simulink model "gmp_pmsm_sensored_nonlinear_sil_mdl_2022b"  (R2022b)
settings: Solver=VariableStepAuto  StartTime=0.0  StopTime=10  RelTol=1e-3
model workspace (MAT data in the model file):
  B = 0
  BW_i = 800
  Flux_t = 0.12
  IQ24 = Simulink.NumericType
  IQ24.DataTypeMode = 'Fixed-point: binary point scaling'
  IQ24.SignednessBool = 1
  IQ24.WordLength = 32
  IQ24.FixedExponent = -16
  IQ24.SlopeAdjustmentFactor = 1
  IQ24.Bias = 0
  IQ24.DataTypeOverride = 'Inherit'
  IQ24.IsAlias = 0
  IQ24.DataScope = 'Auto'
  J = 0.018
  K_d = 3.72061852168
  K_m = 0.128242020589
  K_u = 0.00236407598332
  Ki_id = 0.001
  Ki_iq = 1
  Ki_n = 25225.1136556
  Kp_id = 1e-05
  Kp_iq = 5e-05
  Kp_n = 12.6125568278
  Ld_t = 0.00303
  Lq_t = 0.02019
  Max_p = 0.006000830667
  P = 2
  RLS_ini_a = 1000000
  Rd_mos = 0.01
  Rs = 0.1215
  Rv = 6.4
  T_final = 0
  T_initial = 0
  Tes = [4 7 10 7 4]
  Tf_t = 0.1
  Tm = 0
  Udq_limit = 550
  Var = 0
  Vce0 = 0
  Vd0 = 0
  Vdc = 80
  button = 1
  im_limit = 40
  mean_prd = 10
  position_init = 0.2
  r_ce = 1e-08
  r_d = 1e-08
  sample_prd = 100
  step_time = 0.2
  ts = 6.25e-05
  wc = 3500
libraries: peripheral_utilities x9, spsSeriesRLCBranchLib x6, spsMosfetLib x6, simulink x3, spsVoltageMeasurementLib x2, gmp_sil_core_pack x1, spsPermanentMagnetSynchronousMachineLib x1, spsdq0toabcLib x1, spsFourierLib x1, spsControlledVoltageSourceLib x1, sps_lib x1
(part 1 of 3)
settings Model: SimulationMode=accelerator  Creator=javnson  LastModifiedBy=Lin Minyi

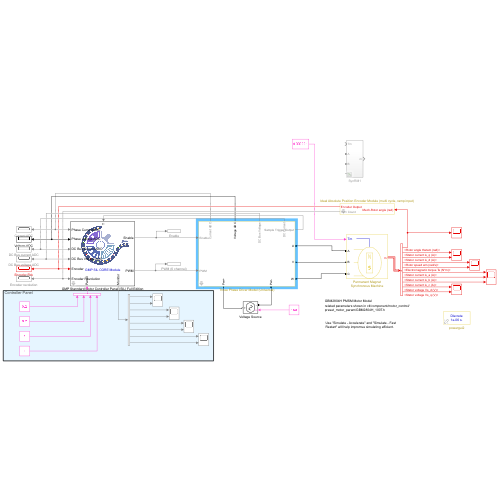
[thumbnail: Simulink's stored preview of the top-level diagram]
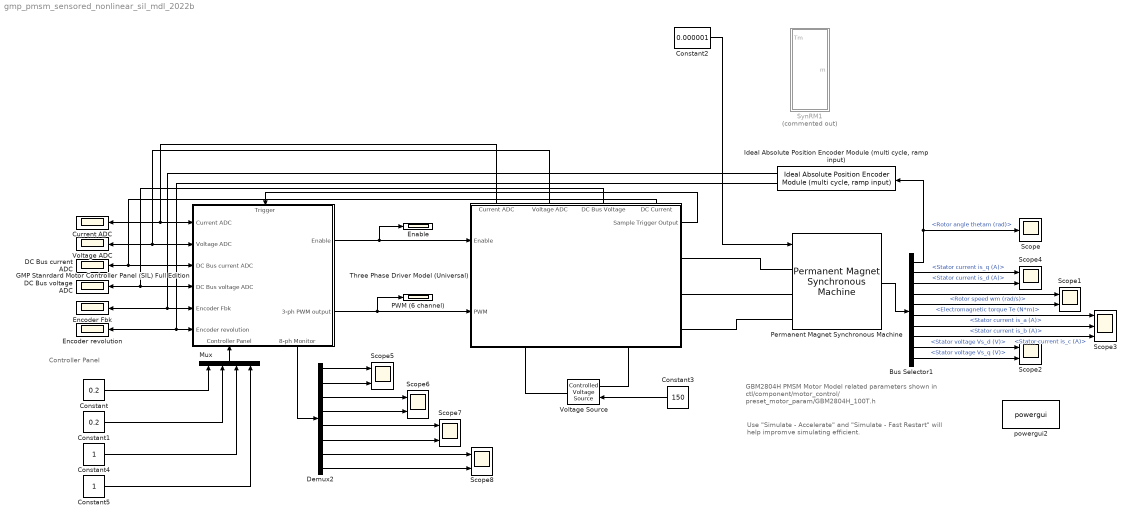
== system gmp_pmsm_sensored_nonlinear_sil_mdl_2022b ==
  note: Use "Simulate - Accelerate" and "Simulate - Fast Restart" will help impromve simulating efficient.
  note: Controller Panel
  note: GBM2804H PMSM Motor Model
      | related parameters shown in ctl/component/motor_control/
      | preset_motor_param/GBM2804H_100T.h
  Bus Selector1 : BusSelector  OutputSignals=Rotor angle thetam (rad),Stator current is_q (A),Stator current is_d (A),Rotor speed wm (rad/s),Electromagnetic torque Te (N*m),Stator current is_a (A),Stator current is_b (A),Stator current is_c (A),Stator voltage Vs_d (V),Stator voltage Vs_q (V)
  Constant : Constant  Value=0.2
  Constant1 : Constant  Value=0.2
  Constant2 : Constant  Value=0.000001
  Constant3 : Constant  Value=150
  Constant4 : Constant
  Constant5 : Constant
  Current ADC : Scope
  DC Bus current ADC : Scope
  DC Bus voltage ADC : Scope
  Demux2 : Demux  Outputs=8
  Enable : Scope
  Encoder Fbk : Scope
  Encoder revolution : Scope
  GMP Stanrdard Motor Controller Panel (SIL) Full Edition : Subsystem  mask(GMP SIL Core for single Motor Controller (full edition)){}
      mask help: This is GMP Motor Simulator port.
      settings: PortSchema="{\"entries\":[{\"content\":{\"sides\":[{\"content\":{\"connectorIds\":[\"In1\",\"In2\",\"In3\",\"In4\",\"In5\",\"In6\"]},\"type\":\"ConnectorPlacement.EquallySpacedRectSide\",\"uuid\":\"45c67bc9-9540-469a-a4ac-1e12eb9acca3\"},{\"content\":{\"connectorIds\":[\"Out1\",\"Out2\"],\"side\":\"RIGHT\"},\"type\":\"ConnectorPlacement.EquallySpacedRectSide\",\"uuid\":\"a17116b4-0460-48ab-8ada-a785da6c5e29\"},{\"content\":{\"connectorIds\":[\"In7\"],\"side\":\"TOP\"},\"type\":\"ConnectorPlacement.EquallySpacedRectSide\",\"uuid\":\"15623697-512e-4e4d-ab51-f53c2346fadb\"},{\"content\":{\"connectorIds\":[\"In8\",\"Out3\"],\"side\":\"BOTTOM\"},\"type\":\"ConnectorPlacement.EquallySpacedRectSide\",\"uuid\":\"47f7968c-22c1-4f3d-97d9-242e9dbf8d30\"}]},\"type\":\"ConnectorPlacement.EquallySpacedConnector\",\"uuid\":\"f369880c-e675-4c1f-982e-a4befb03f503\"}],\"packageUris\":[\"http://schema.mathworks.com/mf0/Connector/R2020b\"],\"version\":\"1.0\"}"
      mask DialogControl ParameterGroupVar Prompt: 参数
      mask Display:
      | image(append(fileparts(which('gmp_simulink_utilities.slx')),'\icon\GMP_Core.png'));
      | color('blue');
      | %text(0.3,0.3,'GMP SIL CORE Module','horizontalAlignment','left','verticalAlignment','bottom');
      | disp('\n\n\n\n\n\n\n\nGMP SIL CORE Module');
      | %text(0,0,'y=a*x^2+b','horizontalAlignment','middle', 'verticalAlignment','bottom');
      | 
      | 
      | module_pos = get_param(gcb, 'Position');
      | width = module_pos(3) - module_pos(1);
      | %rectangle('Position',[module_pos(1),module_pos(2),module_pos(3),module_pos(4)],'FaceColor','r');
      | 
      | color('Black');
      | 
      | port_label('output', 1, 'Enable');
      | port_label('output', 2, 'PWM');
      | port_label('output', 3, 'Monitor');
      | 
      | port_label('input', 1, 'Phase Current ADC');
      | port_label('input', 2, 'Phase Voltage ADC');
      | port_label('input', 3, 'DC Bus Current ADC');
      | port_label('input', 4, 'DC Bus Voltage ADC');
      | port_label('input', 5, 'Encoder');
      | port_label('input', 6, 'Encoder Revolution');
      | port_label('input', 7, 'T');
      | port_label('input', 8, 'Panel');
  "Ideal Absolute Position Encoder Module (multi cycle, ramp input)" : peripheral_utilities/Ideal Absolute Position Encoder Module (multi cycle, ramp input)  ENCODER_BIT=14
      settings: SourceProductName=GMP Utilities Library
  Mux : Mux
  PWM (6 channel) : Scope
  Permanent Magnet Synchronous Machine : spsPermanentMagnetSynchronousMachineLib/Permanent Magnet Synchronous Machine  NbPhases=3  FluxDistribution=Sinusoidal  RotorType=Salient-pole  MechanicalLoad=Torque Tm  PresetModel=No  ShowDetailedParameters=on  MeasurementBus=off  Resistance=Rs  Inductance=8.5e-3  dqInductances=[Ld_t,Lq_t]  La=0.96e-3  MachineConstant=Flux linkage established by magnets (V.s)  Flux=Flux_t  VoltageCst=43.5312  TorqueCst=0.36  Flat=120  Mechanical=[J 1e-8 P 0]  PolePairs=4  InitialConditions=[0, 0, 0, 0]  InitialConditions5ph=[0 0 0 0 0 0]  RefAngle=Aligned with phase A axis (original Park)  IterativeDiscreteModel=Trapezoidal non iterative  TsBlock=-1  TsPowergui=0
  Scope : Scope
  Scope{1..2,4..8} (7 alike) : Scope  NumInputPorts=2
  Scope3 : Scope  NumInputPorts=3
  SynRM1 : Subsystem  Commented=on
  Three Phase Driver Model (Universal) : Subsystem  mask{fswitch=8000, CMP_MAX=6000, Deadband_Upper=48, Deadband_Lower=48, Deadband_us=1, phase_shift=0, R_mosfet_on=0.1, Lon=0, Rd=0.01, Vf=0.3, Rs=1e5, Cs=inf, Rsap=0.005, ADC_GAIN=20, ADC_BIT=12, ADC_REFERENCE=3.3, ADC_BIAS=1.65, ADC_INIT=0, VOLTAGE_ADC_GAIN=0.04049127, VOLTAGE_ADC_BIT=12, VOLTAGE_ADC_REFERENCE=3.3, VOLTAGE_ADC_VOLTAGE=0, VOLTAGE_ADC_INIT=0, VOLTAGE_ADC_CUT_FREQ=1143.4, DCBUS_ADC_GAIN=0.04049127, DCBUS_ADC_BIT=12, DCBUS_ADC_REFERENCE=3.3, DCBUS_ADC_BIAS=0, DCBUS_ADC_INIT=0, DCBUS_CURRENT_ADC_GAIN=1, DCBUS_CURRENT_ADC_BIT=12, DCBUS_CURRENT_ADC_REFERENCE=20, DCBUS_CURRENT_ADC_BIAS=0, DCBUS_CURRENT_ADC_INIT=0}
      mask prompts: DCBUS_CURRENT_ADC_GAIN "DCBUS_ADC_GAIN:"; DCBUS_CURRENT_ADC_BIT "DCBUS_ADC_BIT:"; DCBUS_CURRENT_ADC_REFERENCE "DCBUS_ADC_REFERENCE:"; DCBUS_CURRENT_ADC_BIAS "DCBUS_ADC_BIAS:"; DCBUS_CURRENT_ADC_INIT "DCBUS_ADC_INIT:"
      mask init:
      | calculate_deadband(gcb, 'Deadband_Upper', 'Deadband_Lower',	'CMP_MAX', 'fswitch', 'Deadband_us');
      settings: PortSchema="{\"entries\":[{\"content\":{\"sides\":[{\"content\":{\"connectorIds\":[\"In1\",\"In2\"]},\"type\":\"ConnectorPlacement.EquallySpacedRectSide\",\"uuid\":\"3f4c86ad-0582-4f47-8583-a8af9a7f9adc\"},{\"content\":{\"connectorIds\":[\"Out1\",\"RConn1\",\"RConn2\",\"RConn3\"],\"side\":\"RIGHT\"},\"type\":\"ConnectorPlacement.EquallySpacedRectSide\",\"uuid\":\"ae91f325-3014-4188-9063-296f4d5623fa\"},{\"content\":{\"connectorIds\":[\"Out2\",\"Out3\",\"Out4\",\"Out5\"],\"side\":\"TOP\"},\"type\":\"ConnectorPlacement.EquallySpacedRectSide\",\"uuid\":\"5f2edb36-6849-4a72-b7bd-4d267f120ce4\"},{\"content\":{\"connectorIds\":[\"RConn4\",\"RConn5\"],\"side\":\"BOTTOM\"},\"type\":\"ConnectorPlacement.EquallySpacedRectSide\",\"uuid\":\"79a111ed-6591-4ced-9242-67ea1247c580\"}]},\"type\":\"ConnectorPlacement.EquallySpacedConnector\",\"uuid\":\"8c66eb8e-d25c-472f-a4a5-d1759225ba1c\"}],\"packageUris\":[\"http://schema.mathworks.com/mf0/Connector/R2020b\"],\"version\":\"1.0\"}"
      mask Callback fswitch: calculate_deadband(gcb, 'Deadband_Upper', 'Deadband_Lower',	'CMP_MAX', 'fswitch', 'Deadband_us');
      mask Callback CMP_MAX: calculate_deadband(gcb, 'Deadband_Upper', 'Deadband_Lower',	'CMP_MAX', 'fswitch', 'Deadband_us');
      mask Callback Deadband_Upper: calculate_deadband(gcb, 'Deadband_Upper', 'Deadband_Lower',	'CMP_MAX', 'fswitch', 'Deadband_us');
      mask Callback Deadband_Lower: calculate_deadband(gcb, 'Deadband_Upper', 'Deadband_Lower',	'CMP_MAX', 'fswitch', 'Deadband_us');
      mask DialogControl DescGroupVar Prompt: Three Phases Bridge Peripheral(3-shunt sample)
      mask DialogControl Control21 Prompt: GMP CTL Simulink Utilities: virtual peripherals
      mask DialogControl DescTextVar Prompt: This module provide a ideal 3-phases bridge peripheral.
      mask DialogControl Container4 Prompt: PWM config
      mask DialogControl ParameterGroupVar Prompt: PWM parameters
      mask DialogControl Control2 Prompt: PWM Frequency (Hz):
      mask DialogControl Control4 Prompt: Full Scale PWM Compare value:
      mask DialogControl Control5 Prompt: Deadband Range Set (CMP Value):
      mask DialogControl Control6 Prompt: Deadband time: DEADBAND_CMP/2/CMP_MAX/fswitch
      mask DialogControl Control22 Prompt: Calculated Deadband, us
      mask DialogControl Control20 Prompt: Initial Phase shift:
      mask DialogControl Container5 Prompt: MOSFET config
      mask DialogControl Container7 Prompt: MOSFET parameters
      mask DialogControl Control7 Prompt: Rds(on), unit Ohm
      mask DialogControl Control8 Prompt: Internal diode inducctance, unit H
      mask DialogControl Control9 Prompt: Internal diode resistance Rd, unit Ohm
      mask DialogControl Control10 Prompt: Internal diode forward voltage Vf, unit V
      mask DialogControl Control11 Prompt: Snubber resistance Rs, unit ohm
      mask DialogControl Control12 Prompt: Snubber Capacitance Cs, unit F
      mask DialogControl Container6 Prompt: 3-shunt Current Sample
      mask DialogControl Control13 Prompt: ADC(p.u.) = (real_voltage * ADC_GAIN + ADC_BIAS)/ADC_REFERENCE
      mask DialogControl Control15 Prompt: Shunt Smaple Res, unit Ohm
      mask DialogControl Control14 Prompt: ADC Voltage Gain (Scale Factor):
      mask DialogControl Control16 Prompt: ADC resolution:
      mask DialogControl Control17 Prompt: ADC reference Voltage(V)
      mask DialogControl Control18 Prompt: ADC Bias Voltage(V)
      mask DialogControl Control19 Prompt: ADC Initial Voltage Output (V):
      mask DialogControl Container9 Prompt: 3-shunt Voltage Sample
      mask DialogControl Control34 Prompt: ADC Voltage Gain (Scale Factor):
      mask DialogControl Control23 Prompt: ADC resolution:
      mask DialogControl Control24 Prompt: ADC reference voltage (V), when VOLTAGE_ADC_GAIN = 1, ADC_REF = ADC Full scale
      mask DialogControl Control25 Prompt: ADC Bias Voltage (V):
      mask DialogControl Control26 Prompt: ADC Initial Voltage Output (V):
      mask DialogControl Control27 Prompt: Voltage Filter cut frequency (Hz):
      mask DialogControl Control28 Prompt: Generally, this value less than switch frequency / 10, greater than motor normal frequency * 3
      mask DialogControl Container10 Prompt: DC Bus Voltage Sample
      mask DialogControl Control29 Prompt: ADC Voltage Gain (Scale Factor):
      mask DialogControl Control30 Prompt: ADC resolution:
      mask DialogControl Control32 Prompt: ADC reference voltage (V), when VOLTAGE_ADC_GAIN = 1, ADC_REF = ADC Full scale
      mask DialogControl Control31 Prompt: ADC Bias Voltage (V):
      mask DialogControl Control33 Prompt: ADC Initial Voltage Output (V):
      mask DialogControl Container13 Prompt: DC Bus Current Sample
      mask DialogControl Control29_copy_copy Prompt: ADC Current Gain (Scale Factor):
      mask DialogControl Control30_copy_copy Prompt: ADC resolution:
      mask DialogControl Control32_copy_copy Prompt: ADC reference current (A), when VOLTAGE_ADC_GAIN = 1, ADC_REF = ADC Full scale
      mask DialogControl Control31_copy Prompt: ADC Bias Current (A):
      mask DialogControl Control33_copy Prompt: ADC Initial Current Output (A):
  Voltage ADC : Scope
  Voltage Source : spsControlledVoltageSourceLib/Controlled Voltage Source  Initialize=on  Source_Type=AC  Amplitude=0  Phase=0  Frequency=0  Measurements=None
  powergui2 : sps_lib/powergui  Priority=1  SimulationMode=Discrete  SampleTime=1e-6  frequency=60  Iterations=50  frequencyindice=0  Pbase=100e6  ErrMax=1e-4  UnitsV=kV  UnitsW=MW  buscounter=0  FunctionMessages=off  echomessages=off  EnableUseOfTLC=off  CurrentSourceSwitches=off  DisableSnubberDevices=off  DisableRonSwitches=off  DisableVfSwitches=off  DisplayEquations=off  AutomaticDiscreteSolvers=off  SolverType=Tustin/Backward Euler (TBE)  Interpol=off  ExternalGateDelay=off  methode=off  Ts=100  x0status=blocks  SPID=on  SwTol=0  HookPort=off  NonlinearTolerance=1e-4  nMaxIteration=100  ContinueOnMaxIteration=off  RestoreLinks=warning  ResistiveCurrentMeasurement=off  Frange=[0:2:500]  Ylog=off  Xlog=on  ShowGrid=off  save=off  variable=ZData  structure=0  ZoomFFT=off  StartTime=0.0  cycles=1  DisplayStyle=1  fundamental=60  FreqAxis=off  MaxFrequency=1000  frequencyindicesteady=1  RmsSteady=1  display=off
  wires:
  GMP Stanrdard Motor Controller Panel (SIL) Full Edition/1(Enable) -> Three Phase Driver Model (Universal)/1(Enable), Enable/1
  GMP Stanrdard Motor Controller Panel (SIL) Full Edition/2(3-ph PWM output) -> PWM (6 channel)/1, Three Phase Driver Model (Universal)/2(PWM)
  Constant2/1 -> Permanent Magnet Synchronous Machine/1
  Three Phase Driver Model (Universal)/1(Sample Trigger Output) -> GMP Stanrdard Motor Controller Panel (SIL) Full Edition/7(Trigger)
  Three Phase Driver Model (Universal)/2(Current ADC) -> GMP Stanrdard Motor Controller Panel (SIL) Full Edition/1(Current ADC), Current ADC/1
  Three Phase Driver Model (Universal)/3(Voltage ADC) -> GMP Stanrdard Motor Controller Panel (SIL) Full Edition/2(Voltage ADC), Voltage ADC/1
  Three Phase Driver Model (Universal)/4(DC Bus Voltage) -> DC Bus voltage ADC/1, GMP Stanrdard Motor Controller Panel (SIL) Full Edition/4(DC Bus voltage ADC)
  Permanent Magnet Synchronous Machine/1 -> Bus Selector1/1
  Bus Selector1/1 -> "Ideal Absolute Position Encoder Module (multi cycle, ramp input)"/1, Scope/1  "<Rotor angle thetam (rad)>"
  "Ideal Absolute Position Encoder Module (multi cycle, ramp input)"/1 -> Encoder Fbk/1, GMP Stanrdard Motor Controller Panel (SIL) Full Edition/5(Encoder Fbk)
  Bus Selector1/3 -> Scope4/2  "<Stator current is_d (A)>"
  Bus Selector1/2 -> Scope4/1  "<Stator current is_q (A)>"
  Constant3/1 -> Voltage Source/1
  Demux2/4 -> Scope6/2
  Demux2/3 -> Scope6/1
  Demux2/2 -> Scope5/2
  Demux2/1 -> Scope5/1
  GMP Stanrdard Motor Controller Panel (SIL) Full Edition/3(8-ph Monitor) -> Demux2/1
  Bus Selector1/4 -> Scope1/1  "<Rotor speed wm (rad/s)>"
  Bus Selector1/5 -> Scope1/2  "<Electromagnetic torque Te (N*m)>"
  "Ideal Absolute Position Encoder Module (multi cycle, ramp input)"/2 -> Encoder revolution/1, GMP Stanrdard Motor Controller Panel (SIL) Full Edition/6(Encoder revolution)
  Mux/1 -> GMP Stanrdard Motor Controller Panel (SIL) Full Edition/8(Controller Panel)
  Constant/1 -> Mux/1
  Constant1/1 -> Mux/2
  Constant4/1 -> Mux/3
  Constant5/1 -> Mux/4
  Demux2/5 -> Scope7/1
  Demux2/6 -> Scope7/2
  Demux2/7 -> Scope8/1
  Demux2/8 -> Scope8/2
  Three Phase Driver Model (Universal)/5(DC Current) -> DC Bus current ADC/1, GMP Stanrdard Motor Controller Panel (SIL) Full Edition/3(DC Bus current ADC)
  Bus Selector1/9 -> Scope2/1  "<Stator voltage Vs_d (V)>"
  Bus Selector1/10 -> Scope2/2  "<Stator voltage Vs_q (V)>"
  Bus Selector1/6 -> Scope3/1  "<Stator current is_a (A)>"
  Bus Selector1/7 -> Scope3/2  "<Stator current is_b (A)>"
  Bus Selector1/8 -> Scope3/3  "<Stator current is_c (A)>"
  connections:
  Permanent Magnet Synchronous Machine/LConn2 -- Three Phase Driver Model (Universal)/RConn2
  Three Phase Driver Model (Universal)/RConn3 -- Permanent Magnet Synchronous Machine/LConn3
  Permanent Magnet Synchronous Machine/LConn1 -- Three Phase Driver Model (Universal)/RConn1
  Three Phase Driver Model (Universal)/RConn5 -- Voltage Source/LConn1
  Three Phase Driver Model (Universal)/RConn4 -- Voltage Source/RConn1

== system gmp_pmsm_sensored_nonlinear_sil_mdl_2022b/GMP Stanrdard Motor Controller Panel (SIL) Full Edition ==
  Current ADC : Inport
  Voltage ADC : Inport  Port=2
  DC Bus current ADC : Inport  Port=3
  DC Bus voltage ADC : Inport  Port=4
  Encoder Fbk : Inport  Port=5
  Encoder revolution : Inport  Port=6
  Trigger : Inport  Port=7
  Controller Panel : Inport  Port=8
  GMP SIL Core With trigger : Subsystem
  Simulation Time : Clock
  Enable : Outport
  3-ph PWM output : Outport  Port=2
  8-ph Monitor : Outport  Port=3
  wires:
  Encoder Fbk/1 -> GMP SIL Core With trigger/6(Encoder Fbk)
  Encoder revolution/1 -> GMP SIL Core With trigger/7(Encoder revolution)
  GMP SIL Core With trigger/2(3-ph PWM output) -> 3-ph PWM output/1
  Simulation Time/1 -> GMP SIL Core With trigger/1(time)
  GMP SIL Core With trigger/1(Enable) -> Enable/1
  Voltage ADC/1 -> GMP SIL Core With trigger/3(Voltage ADC)
  Current ADC/1 -> GMP SIL Core With trigger/2(Current ADC)
  GMP SIL Core With trigger/3(8-ph Monitor) -> 8-ph Monitor/1
  DC Bus current ADC/1 -> GMP SIL Core With trigger/4(DC Bus current ADC)
  Trigger/1 -> GMP SIL Core With trigger/Trigger
  DC Bus voltage ADC/1 -> GMP SIL Core With trigger/5(DC bus voltage ADC)
  Controller Panel/1 -> GMP SIL Core With trigger/8(Panel Input)

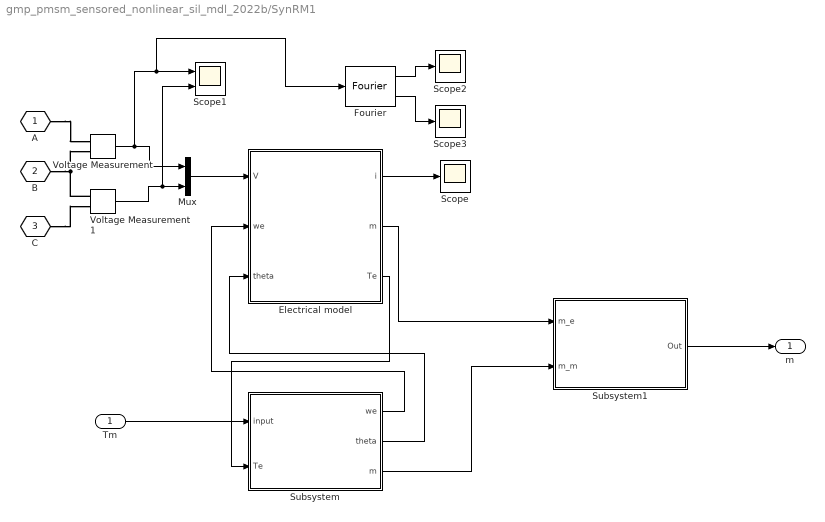
== system gmp_pmsm_sensored_nonlinear_sil_mdl_2022b/SynRM1 ==
  Tm : Inport
  Electrical model : Subsystem
  Fourier : spsFourierLib/Fourier  Freq=100  n=1  InInit=[0, 0]  Ts=0
  Mux : Mux  Inputs=2
  Scope : Scope
  Scope1 : Scope  NumInputPorts=2
  Scope2 : Scope
  Scope3 : Scope
  Subsystem : Subsystem
  Subsystem1 : Subsystem
  Voltage Measurement : spsVoltageMeasurementLib/Voltage Measurement  PhasorSimulation=off  OutputType=Complex  PSBequivalent=0
  Voltage Measurement1 : spsVoltageMeasurementLib/Voltage Measurement  PhasorSimulation=off  OutputType=Complex  PSBequivalent=0
  A : PMIOPort  Side=Left
  B : PMIOPort  Port=2  Side=Left
  C : PMIOPort  Port=3  Side=Left
  m : Outport  VectorParamsAs1DForOutWhenUnconnected=off
  wires:
  Subsystem/3(m) -> Subsystem1/2(m_m)
  Subsystem/1(we) -> Electrical model/2(we)
  Mux/1 -> Electrical model/1(V)
  Subsystem/2(theta) -> Electrical model/3(theta)
  Electrical model/3(Te) -> Subsystem/2(Te)
  Subsystem1/1(Out) -> m/1
  Electrical model/1(i) -> Scope/1
  Electrical model/2(m) -> Subsystem1/1(m_e)
  Tm/1 -> Subsystem/1(input)
  Voltage Measurement/1 -> Fourier/1, Scope1/1, Mux/1
  Voltage Measurement1/1 -> Scope1/2, Mux/2
  Fourier/1 -> Scope2/1
  Fourier/2 -> Scope3/1
  connections:
  C/RConn1 -- Voltage Measurement1/LConn2
  A/RConn1 -- Voltage Measurement/LConn1
  B/RConn1 -- Voltage Measurement1/LConn1 -- Voltage Measurement/LConn2

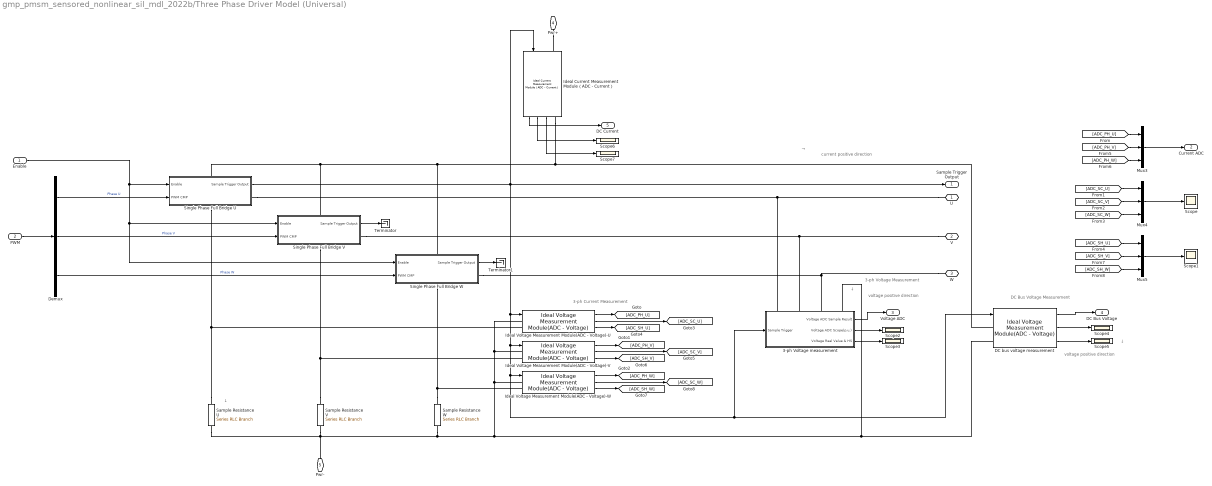
== system gmp_pmsm_sensored_nonlinear_sil_mdl_2022b/Three Phase Driver Model (Universal) ==
  note: 3-ph Current Measurement
  note: →
  note: current positive direction
  note: ↓
  note: voltage positive direction
  note: ↓
  note: 3-ph Voltage Measurement
  note: DC Bus Voltage Measurement
  note: ↓
  note: voltage positive direction
  Enable : Inport
  PWM : Inport  Port=2
  3-ph Voltage measurement : Subsystem  AncestorBlock=peripheral_utilities/Three Phases Voltage (ph-gnd) Measurement with Filter  mask{ADC_GAIN=VOLTAGE_ADC_GAIN, ADC_BIT=VOLTAGE_ADC_BIT, ADC_REFERENCE=VOLTAGE_ADC_REFERENCE, ADC_BIAS=VOLTAGE_ADC_VOLTAGE, ADC_INIT=VOLTAGE_ADC_INIT, cut_frequency=VOLTAGE_ADC_CUT_FREQ}
      settings: PortSchema="{\"entries\":[{\"content\":{\"sides\":[{\"content\":{\"connectorIds\":[\"In1\"]},\"type\":\"ConnectorPlacement.EquallySpacedRectSide\",\"uuid\":\"ae4f4612-c092-4fa0-8a43-5c9e823110e3\"},{\"content\":{\"connectorIds\":[\"Out1\",\"Out2\",\"Out3\"],\"side\":\"RIGHT\"},\"type\":\"ConnectorPlacement.EquallySpacedRectSide\",\"uuid\":\"6db15ef0-d33a-4775-b4e6-14a566796673\"},{\"content\":{\"connectorIds\":[\"LConn1\",\"LConn2\",\"LConn3\",\"LConn4\"],\"side\":\"TOP\"},\"type\":\"ConnectorPlacement.EquallySpacedRectSide\",\"uuid\":\"cfddd664-59f3-497b-b33e-fe832fe7a7bd\"}]},\"type\":\"ConnectorPlacement.EquallySpacedConnector\",\"uuid\":\"5bacf0ad-0c4a-4f47-a242-d8a476ab7f52\"}],\"packageUris\":[\"http://schema.mathworks.com/mf0/Connector/R2020b\"],\"version\":\"1.0\"}"
      mask DialogControl DescGroupVar Prompt: 3 phases Voltage Sample ADC Model
      mask DialogControl Control10 Prompt: GMP CTL Simulink Utilities: virtual peripherals
      mask DialogControl DescTextVar Prompt: This is a ideal Voltage Measurement Module.
      mask DialogControl Control2 Prompt: ADC(p.u.) = (real_voltage * ADC_GAIN + ADC_BIAS)/ADC_REFERENCE
      mask DialogControl ParameterGroupVar Prompt: parameters:
      mask DialogControl Control3 Prompt: ADC Voltage Gain (Scale Factor):
      mask DialogControl Control4 Prompt: ADC resolution:
      mask DialogControl Control5 Prompt: ADC reference Voltage (V), when ADC_GAIN=1, ADC_REF = ADC full scale
      mask DialogControl Control6 Prompt: ADC Bias Voltage(V)
      mask DialogControl Control7 Prompt: ADC Initial Voltage Output (V):
      mask DialogControl Control8 Prompt: Voltage Filter cut frequency (Hz):
      mask DialogControl Control9 Prompt: Generally, this value less than switch frequency / 10, greater than motor normal frequency * 3
  DC bus voltage measurement : peripheral_utilities/Ideal Voltage Measurement Module(ADC - Voltage)  ADC_GAIN=DCBUS_ADC_GAIN  ADC_BIT=DCBUS_ADC_BIT  ADC_REFERENCE=DCBUS_ADC_REFERENCE  ADC_BIAS=DCBUS_ADC_BIAS  ADC_INIT=DCBUS_ADC_INIT
      settings: SourceProductName=GMP Utilities Library
  Demux : Demux  Outputs=3
  Ideal Current Measurement Module（ADC - Current） : peripheral_utilities/Ideal Current Measurement Module（ADC - Current）  ADC_GAIN=DCBUS_CURRENT_ADC_GAIN  ADC_BIT=DCBUS_CURRENT_ADC_BIT  ADC_REFERENCE=DCBUS_CURRENT_ADC_REFERENCE  ADC_BIAS=DCBUS_CURRENT_ADC_BIAS  ADC_INIT=DCBUS_CURRENT_ADC_INIT
      settings: SourceProductName=GMP Utilities Library
  Ideal Voltage Measurement Module(ADC - Voltage)-U : peripheral_utilities/Ideal Voltage Measurement Module(ADC - Voltage)  ADC_GAIN=ADC_GAIN  ADC_BIT=ADC_BIT  ADC_REFERENCE=ADC_REFERENCE  ADC_BIAS=ADC_BIAS  ADC_INIT=ADC_INIT
      settings: SourceProductName=GMP Utilities Library
  Ideal Voltage Measurement Module(ADC - Voltage)-V : peripheral_utilities/Ideal Voltage Measurement Module(ADC - Voltage)  ADC_GAIN=ADC_GAIN  ADC_BIT=ADC_BIT  ADC_REFERENCE=ADC_REFERENCE  ADC_BIAS=ADC_BIAS  ADC_INIT=ADC_INIT
      settings: SourceProductName=GMP Utilities Library
  Ideal Voltage Measurement Module(ADC - Voltage)-W : peripheral_utilities/Ideal Voltage Measurement Module(ADC - Voltage)  ADC_GAIN=ADC_GAIN  ADC_BIT=ADC_BIT  ADC_REFERENCE=ADC_REFERENCE  ADC_BIAS=ADC_BIAS  ADC_INIT=ADC_INIT
      settings: SourceProductName=GMP Utilities Library
  Mux3 : Mux  Inputs=3
  Mux4 : Mux  Inputs=3
  Mux5 : Mux  Inputs=3
  Sample Resistance U : spsSeriesRLCBranchLib/Series RLC Branch  LConnTagsString=__new0  RConnTagsString=__new0  BranchType=R  Resistance=Rsap  Inductance=1e-3  SetiL0=off  InitialCurrent=0  Capacitance=1e-6  Setx0=off  InitialVoltage=0  Measurements=None
  Sample Resistance V : spsSeriesRLCBranchLib/Series RLC Branch  LConnTagsString=__new0  RConnTagsString=__new0  BranchType=R  Resistance=Rsap  Inductance=1e-3  SetiL0=off  InitialCurrent=0  Capacitance=1e-6  Setx0=off  InitialVoltage=0  Measurements=None
  Sample Resistance W : spsSeriesRLCBranchLib/Series RLC Branch  LConnTagsString=__new0  RConnTagsString=__new0  BranchType=R  Resistance=Rsap  Inductance=1e-3  SetiL0=off  InitialCurrent=0  Capacitance=1e-6  Setx0=off  InitialVoltage=0  Measurements=None
  Scope{,1..7} (8 alike) : Scope
  Single Phase Full Bridge U : Subsystem  mask{fswitch=fswitch, CMP_MAX=CMP_MAX, Deadband_Upper=Deadband_Upper, Deadband_Lower=Deadband_Lower, Deadband_us=NaN, phase_shift=phase_shift, R_mosfet_on=R_mosfet_on, Lon=Lon, Rd=Rd, Vf=Vf, Rs=Rs, Cs=Cs}
      mask init:
      | calculate_deadband(gcb, 'Deadband_Upper', 'Deadband_Lower',	'CMP_MAX', 'fswitch', 'Deadband_us');
      settings: PortSchema="{\"entries\":[{\"content\":{\"sides\":[{\"content\":{\"connectorIds\":[\"In1\",\"In2\"]},\"type\":\"ConnectorPlacement.EquallySpacedRectSide\",\"uuid\":\"20beeabc-b0ca-4337-b227-c7f02abd15d8\"},{\"content\":{\"connectorIds\":[\"Out1\",\"RConn1\"],\"side\":\"RIGHT\"},\"type\":\"ConnectorPlacement.EquallySpacedRectSide\",\"uuid\":\"a7923383-ac55-4621-ad1d-4d067c1fb84d\"},{\"content\":{\"connectorIds\":[\"LConn1\"],\"side\":\"TOP\"},\"type\":\"ConnectorPlacement.EquallySpacedRectSide\",\"uuid\":\"661bf0ae-1c96-4de8-96aa-28c06a0a56db\"},{\"content\":{\"connectorIds\":[\"RConn2\"],\"side\":\"BOTTOM\"},\"type\":\"ConnectorPlacement.EquallySpacedRectSide\",\"uuid\":\"fc2f6321-5787-4e1a-b5a2-65ed34db36b5\"}]},\"type\":\"ConnectorPlacement.EquallySpacedConnector\",\"uuid\":\"e2219b16-0a50-43ef-8183-c55a35d5a2a0\"}],\"packageUris\":[\"http://schema.mathworks.com/mf0/Connector/R2020b\"],\"version\":\"1.0\"}"
      mask Callback fswitch: calculate_deadband(gcb, 'Deadband_Upper', 'Deadband_Lower',	'CMP_MAX', 'fswitch', 'Deadband_us');
      mask Callback CMP_MAX: calculate_deadband(gcb, 'Deadband_Upper', 'Deadband_Lower',	'CMP_MAX', 'fswitch', 'Deadband_us');
      mask Callback Deadband_Upper: calculate_deadband(gcb, 'Deadband_Upper', 'Deadband_Lower',	'CMP_MAX', 'fswitch', 'Deadband_us');
      mask Callback Deadband_Lower: calculate_deadband(gcb, 'Deadband_Upper', 'Deadband_Lower',	'CMP_MAX', 'fswitch', 'Deadband_us');
      mask DialogControl DescGroupVar Prompt: Half Bridge With PWM Module
      mask DialogControl Control14 Prompt: GMP CTL Simulink Utilities: virtual peripherals
      mask DialogControl DescTextVar Prompt: This module provide a PWM (with deadband), and a MOSFET half bridge.
      mask DialogControl Container5 Prompt: PWM Modulator
      mask DialogControl ParameterGroupVar Prompt: PWM module parameters
      mask DialogControl Control2 Prompt: PWM Frequency (Hz):
      mask DialogControl Control3 Prompt: Full Scale PWM Compare value:
      mask DialogControl Control4 Prompt: (whole period is 2 * CMP_MAX ticks)
      mask DialogControl Control5 Prompt: Deadband Range Set (CMP Value):
      mask DialogControl Control6 Prompt: Single side deadband time: DEADBAND_CMP/2/CMP_MAX/fswitch
      mask DialogControl Control15 Prompt: Calculated Deadband, us
      mask DialogControl Control13 Prompt: Initial Phase Shift, unit rad
      mask DialogControl Container6 Prompt: MOSFET
      mask DialogControl Container3 Prompt: MOSFET parameters
      mask DialogControl Control7 Prompt: Rds(on), unit Ohm
      mask DialogControl Control8 Prompt: Internal diode inducctance, unit H
      mask DialogControl Control9 Prompt: Internal diode resistance Rd, unit Ohm
      mask DialogControl Control10 Prompt: Internal diode forward voltage Vf, unit V
      mask DialogControl Control11 Prompt: Snubber resistance Rs, unit ohm
      mask DialogControl Control12 Prompt: Snubber Capacitance Cs, unit F
  Single Phase Full Bridge V : Subsystem  mask{fswitch=fswitch, CMP_MAX=CMP_MAX, Deadband_Upper=Deadband_Upper, Deadband_Lower=Deadband_Lower, Deadband_us=NaN, phase_shift=phase_shift, R_mosfet_on=R_mosfet_on, Lon=Lon, Rd=Rd, Vf=Vf, Rs=Rs, Cs=Cs}
      mask init:
      | calculate_deadband(gcb, 'Deadband_Upper', 'Deadband_Lower',	'CMP_MAX', 'fswitch', 'Deadband_us');
      settings: PortSchema="{\"entries\":[{\"content\":{\"sides\":[{\"content\":{\"connectorIds\":[\"In1\",\"In2\"]},\"type\":\"ConnectorPlacement.EquallySpacedRectSide\",\"uuid\":\"20beeabc-b0ca-4337-b227-c7f02abd15d8\"},{\"content\":{\"connectorIds\":[\"Out1\",\"RConn1\"],\"side\":\"RIGHT\"},\"type\":\"ConnectorPlacement.EquallySpacedRectSide\",\"uuid\":\"a7923383-ac55-4621-ad1d-4d067c1fb84d\"},{\"content\":{\"connectorIds\":[\"LConn1\"],\"side\":\"TOP\"},\"type\":\"ConnectorPlacement.EquallySpacedRectSide\",\"uuid\":\"661bf0ae-1c96-4de8-96aa-28c06a0a56db\"},{\"content\":{\"connectorIds\":[\"RConn2\"],\"side\":\"BOTTOM\"},\"type\":\"ConnectorPlacement.EquallySpacedRectSide\",\"uuid\":\"fc2f6321-5787-4e1a-b5a2-65ed34db36b5\"}]},\"type\":\"ConnectorPlacement.EquallySpacedConnector\",\"uuid\":\"e2219b16-0a50-43ef-8183-c55a35d5a2a0\"}],\"packageUris\":[\"http://schema.mathworks.com/mf0/Connector/R2020b\"],\"version\":\"1.0\"}"
      mask Callback fswitch: calculate_deadband(gcb, 'Deadband_Upper', 'Deadband_Lower',	'CMP_MAX', 'fswitch', 'Deadband_us');
      mask Callback CMP_MAX: calculate_deadband(gcb, 'Deadband_Upper', 'Deadband_Lower',	'CMP_MAX', 'fswitch', 'Deadband_us');
      mask Callback Deadband_Upper: calculate_deadband(gcb, 'Deadband_Upper', 'Deadband_Lower',	'CMP_MAX', 'fswitch', 'Deadband_us');
      mask Callback Deadband_Lower: calculate_deadband(gcb, 'Deadband_Upper', 'Deadband_Lower',	'CMP_MAX', 'fswitch', 'Deadband_us');
      mask DialogControl DescGroupVar Prompt: Half Bridge With PWM Module
      mask DialogControl Control14 Prompt: GMP CTL Simulink Utilities: virtual peripherals
      mask DialogControl DescTextVar Prompt: This module provide a PWM (with deadband), and a MOSFET half bridge.
      mask DialogControl Container5 Prompt: PWM Modulator
      mask DialogControl ParameterGroupVar Prompt: PWM module parameters
      mask DialogControl Control2 Prompt: PWM Frequency (Hz):
      mask DialogControl Control3 Prompt: Full Scale PWM Compare value:
      mask DialogControl Control4 Prompt: (whole period is 2 * CMP_MAX ticks)
      mask DialogControl Control5 Prompt: Deadband Range Set (CMP Value):
      mask DialogControl Control6 Prompt: Single side deadband time: DEADBAND_CMP/2/CMP_MAX/fswitch
      mask DialogControl Control15 Prompt: Calculated Deadband, us
      mask DialogControl Control13 Prompt: Initial Phase Shift, unit rad
      mask DialogControl Container6 Prompt: MOSFET
      mask DialogControl Container3 Prompt: MOSFET parameters
      mask DialogControl Control7 Prompt: Rds(on), unit Ohm
      mask DialogControl Control8 Prompt: Internal diode inducctance, unit H
      mask DialogControl Control9 Prompt: Internal diode resistance Rd, unit Ohm
      mask DialogControl Control10 Prompt: Internal diode forward voltage Vf, unit V
      mask DialogControl Control11 Prompt: Snubber resistance Rs, unit ohm
      mask DialogControl Control12 Prompt: Snubber Capacitance Cs, unit F
  Single Phase Full Bridge W : Subsystem  mask{fswitch=fswitch, CMP_MAX=CMP_MAX, Deadband_Upper=Deadband_Upper, Deadband_Lower=Deadband_Lower, Deadband_us=NaN, phase_shift=phase_shift, R_mosfet_on=R_mosfet_on, Lon=Lon, Rd=Rd, Vf=Vf, Rs=Rs, Cs=Cs}
      mask init:
      | calculate_deadband(gcb, 'Deadband_Upper', 'Deadband_Lower',	'CMP_MAX', 'fswitch', 'Deadband_us');
      settings: PortSchema="{\"entries\":[{\"content\":{\"sides\":[{\"content\":{\"connectorIds\":[\"In1\",\"In2\"]},\"type\":\"ConnectorPlacement.EquallySpacedRectSide\",\"uuid\":\"20beeabc-b0ca-4337-b227-c7f02abd15d8\"},{\"content\":{\"connectorIds\":[\"Out1\",\"RConn1\"],\"side\":\"RIGHT\"},\"type\":\"ConnectorPlacement.EquallySpacedRectSide\",\"uuid\":\"a7923383-ac55-4621-ad1d-4d067c1fb84d\"},{\"content\":{\"connectorIds\":[\"LConn1\"],\"side\":\"TOP\"},\"type\":\"ConnectorPlacement.EquallySpacedRectSide\",\"uuid\":\"661bf0ae-1c96-4de8-96aa-28c06a0a56db\"},{\"content\":{\"connectorIds\":[\"RConn2\"],\"side\":\"BOTTOM\"},\"type\":\"ConnectorPlacement.EquallySpacedRectSide\",\"uuid\":\"fc2f6321-5787-4e1a-b5a2-65ed34db36b5\"}]},\"type\":\"ConnectorPlacement.EquallySpacedConnector\",\"uuid\":\"e2219b16-0a50-43ef-8183-c55a35d5a2a0\"}],\"packageUris\":[\"http://schema.mathworks.com/mf0/Connector/R2020b\"],\"version\":\"1.0\"}"
      mask Callback fswitch: calculate_deadband(gcb, 'Deadband_Upper', 'Deadband_Lower',	'CMP_MAX', 'fswitch', 'Deadband_us');
      mask Callback CMP_MAX: calculate_deadband(gcb, 'Deadband_Upper', 'Deadband_Lower',	'CMP_MAX', 'fswitch', 'Deadband_us');
      mask Callback Deadband_Upper: calculate_deadband(gcb, 'Deadband_Upper', 'Deadband_Lower',	'CMP_MAX', 'fswitch', 'Deadband_us');
      mask Callback Deadband_Lower: calculate_deadband(gcb, 'Deadband_Upper', 'Deadband_Lower',	'CMP_MAX', 'fswitch', 'Deadband_us');
      mask DialogControl DescGroupVar Prompt: Half Bridge With PWM Module
      mask DialogControl Control14 Prompt: GMP CTL Simulink Utilities: virtual peripherals
      mask DialogControl DescTextVar Prompt: This module provide a PWM (with deadband), and a MOSFET half bridge.
      mask DialogControl Container5 Prompt: PWM Modulator
      mask DialogControl ParameterGroupVar Prompt: PWM module parameters
      mask DialogControl Control2 Prompt: PWM Frequency (Hz):
      mask DialogControl Control3 Prompt: Full Scale PWM Compare value:
      mask DialogControl Control4 Prompt: (whole period is 2 * CMP_MAX ticks)
      mask DialogControl Control5 Prompt: Deadband Range Set (CMP Value):
      mask DialogControl Control6 Prompt: Single side deadband time: DEADBAND_CMP/2/CMP_MAX/fswitch
      mask DialogControl Control15 Prompt: Calculated Deadband, us
      mask DialogControl Control13 Prompt: Initial Phase Shift, unit rad
      mask DialogControl Container6 Prompt: MOSFET
      mask DialogControl Container3 Prompt: MOSFET parameters
      mask DialogControl Control7 Prompt: Rds(on), unit Ohm
      mask DialogControl Control8 Prompt: Internal diode inducctance, unit H
      mask DialogControl Control9 Prompt: Internal diode resistance Rd, unit Ohm
      mask DialogControl Control10 Prompt: Internal diode forward voltage Vf, unit V
      mask DialogControl Control11 Prompt: Snubber resistance Rs, unit ohm
      mask DialogControl Control12 Prompt: Snubber Capacitance Cs, unit F
  Terminator : Terminator
  Terminator1 : Terminator
  U : PMIOPort  Side=Right
  V : PMIOPort  Port=2  Side=Right
  W : PMIOPort  Port=3  Side=Right
  Pwr+ : PMIOPort  Port=4  Side=Right
  Pwr- : PMIOPort  Port=5  Side=Right
  Sample Trigger Output : Outport
  Current ADC : Outport  Port=2
  Voltage ADC : Outport  Port=3
  DC Bus Voltage : Outport  Port=4
  DC Current : Outport  Port=5
  wires:
  Demux/1 -> Single Phase Full Bridge U/2(PWM CMP)  "Phase U"
  Ideal Voltage Measurement Module(ADC - Voltage)-U/1 -> [ADC_PH_U]
  Single Phase Full Bridge V/1(Sample Trigger Output) -> Terminator/1
  Single Phase Full Bridge W/1(Sample Trigger Output) -> Terminator1/1
  Ideal Voltage Measurement Module(ADC - Voltage)-U/2 -> [ADC_SC_U]
  Demux/2 -> Single Phase Full Bridge V/2(PWM CMP)  "Phase V"
  Demux/3 -> Single Phase Full Bridge W/2(PWM CMP)  "Phase W"
  [ADC_PH_V] -> Mux3/2
  [ADC_SC_V] -> Mux4/2
  Ideal Voltage Measurement Module(ADC - Voltage)-U/3 -> [ADC_SH_U]
  Mux3/1 -> Current ADC/1
  Ideal Voltage Measurement Module(ADC - Voltage)-V/1 -> [ADC_PH_V]
  [ADC_SC_U] -> Mux4/1
  [ADC_SH_W] -> Mux5/3
  Mux5/1 -> Scope1/1
  Ideal Voltage Measurement Module(ADC - Voltage)-W/1 -> [ADC_PH_W]
  [ADC_PH_U] -> Mux3/1
  Enable/1 -> Single Phase Full Bridge U/1(Enable), Single Phase Full Bridge W/1(Enable), Single Phase Full Bridge V/1(Enable)
  Mux4/1 -> Scope/1
  Ideal Voltage Measurement Module(ADC - Voltage)-V/3 -> [ADC_SH_V]
  Single Phase Full Bridge U/1(Sample Trigger Output) -> Sample Trigger Output/1, Ideal Current Measurement Module（ADC - Current）/1, Ideal Voltage Measurement Module(ADC - Voltage)-V/1, Ideal Voltage Measurement Module(ADC - Voltage)-W/1, DC bus voltage measurement/1, 3-ph Voltage measurement/1(Sample Trigger), Ideal Voltage Measurement Module(ADC - Voltage)-U/1
  [ADC_SH_U] -> Mux5/1
  Ideal Voltage Measurement Module(ADC - Voltage)-V/2 -> [ADC_SC_V]
  Ideal Voltage Measurement Module(ADC - Voltage)-W/3 -> [ADC_SH_W]
  [ADC_PH_W] -> Mux3/3
  [ADC_SC_W] -> Mux4/3
  [ADC_SH_V] -> Mux5/2
  Ideal Voltage Measurement Module(ADC - Voltage)-W/2 -> [ADC_SC_W]
  3-ph Voltage measurement/1(Voltage ADC Sample Result) -> Voltage ADC/1
  3-ph Voltage measurement/2(Voltage ADC Scope(p.u.)) -> Scope2/1
  3-ph Voltage measurement/3(Voltage Real Value & HS) -> Scope3/1
  DC bus voltage measurement/1 -> DC Bus Voltage/1
  DC bus voltage measurement/2 -> Scope4/1
  DC bus voltage measurement/3 -> Scope5/1
  PWM/1 -> Demux/1
  Ideal Current Measurement Module（ADC - Current）/1 -> DC Current/1
  Ideal Current Measurement Module（ADC - Current）/2 -> Scope6/1
  Ideal Current Measurement Module（ADC - Current）/3 -> Scope7/1
  connections:
  V/RConn1 -- Single Phase Full Bridge V/RConn1 -- 3-ph Voltage measurement/LConn2
  U/RConn1 -- Single Phase Full Bridge U/RConn1 -- 3-ph Voltage measurement/LConn1
  W/RConn1 -- Single Phase Full Bridge W/RConn1 -- 3-ph Voltage measurement/LConn3
  Sample Resistance V/LConn1 -- Single Phase Full Bridge V/RConn2 -- Ideal Voltage Measurement Module(ADC - Voltage)-V/LConn2
  Pwr-/RConn1 -- Sample Resistance U/RConn1 -- Sample Resistance V/RConn1 -- Sample Resistance W/RConn1 -- 3-ph Voltage measurement/LConn4 -- DC bus voltage measurement/LConn2 -- Ideal Voltage Measurement Module(ADC - Voltage)-U/LConn1 -- Ideal Voltage Measurement Module(ADC - Voltage)-V/LConn1 -- Ideal Voltage Measurement Module(ADC - Voltage)-W/LConn1
  Sample Resistance W/LConn1 -- Single Phase Full Bridge W/RConn2 -- Ideal Voltage Measurement Module(ADC - Voltage)-W/LConn2
  Sample Resistance U/LConn1 -- Single Phase Full Bridge U/RConn2 -- Ideal Voltage Measurement Module(ADC - Voltage)-U/LConn2
  Single Phase Full Bridge W/LConn1 -- DC bus voltage measurement/LConn1 -- Ideal Current Measurement Module（ADC - Current）/RConn1 -- Single Phase Full Bridge V/LConn1 -- Single Phase Full Bridge U/LConn1
  Pwr+/RConn1 -- Ideal Current Measurement Module（ADC - Current）/LConn1

== system gmp_pmsm_sensored_nonlinear_sil_mdl_2022b/GMP Stanrdard Motor Controller Panel (SIL) Full Edition/GMP SIL Core With trigger ==
  note: NOTIC:
      | Windows平台下必须设置为正确的内存对齐方式，否则会导致收到的数据乱码！
      | 对于X64的编译方式，默认的内存对齐为8；
      | 对于X86的编译方式，默认的内存对齐为4。
  time : Inport
  Current ADC : Inport  Port=2
  Voltage ADC : Inport  Port=3
  DC Bus current ADC : Inport  Port=4
  DC bus voltage ADC : Inport  Port=5
  Encoder Fbk : Inport  Port=6
  Encoder revolution : Inport  Port=7
  Panel Input : Inport  Port=8
  Trigger : TriggerPort  VariantControl=(inherit)  PortDimensions=1
  GMP SIL Core Module : gmp_sil_core_pack/GMP SIL Core Module  MaskPackedDataTypes={'double','uint32','uint32','uint32','uint32', 'uint32', 'int32', 'double'}  MaskPackedDataSizes={[1],[3],[3],[1],[1], [1], [1], [4]}  MaskUnpackedDataTypes={'double', 'uint32','double'}  MaskUnpackedDataSizes={[1],[3],[8]}  MaskAlignment=1  MaskHostAddr='127.0.0.1'  MaskMsgTxPort=12300  MaskMsgRxPort=12301  MaskCmdTxPort=12302  MaskCmdRxPort=12303
      settings: SourceProductName=GMP Utilities Library
  Enable : Outport
  3-ph PWM output : Outport  Port=2
  8-ph Monitor : Outport  Port=3
  wires:
  Current ADC/1 -> GMP SIL Core Module/2
  Voltage ADC/1 -> GMP SIL Core Module/3
  DC Bus current ADC/1 -> GMP SIL Core Module/4
  time/1 -> GMP SIL Core Module/1
  GMP SIL Core Module/3 -> 8-ph Monitor/1
  GMP SIL Core Module/2 -> 3-ph PWM output/1
  GMP SIL Core Module/1 -> Enable/1
  Encoder Fbk/1 -> GMP SIL Core Module/6
  Encoder revolution/1 -> GMP SIL Core Module/7
  DC bus voltage ADC/1 -> GMP SIL Core Module/5
  Panel Input/1 -> GMP SIL Core Module/8
